simulink model "SlidingModeObserver"  (R2026b)
settings: Solver=VariableStepAuto
undefined symbols (not defined in the file or in its folder): smoCfg
libraries: AngleTracking x1
settings Model: Creator=24322  LastModifiedBy=24322

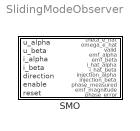
== system SlidingModeObserver ==
  SMO : Subsystem

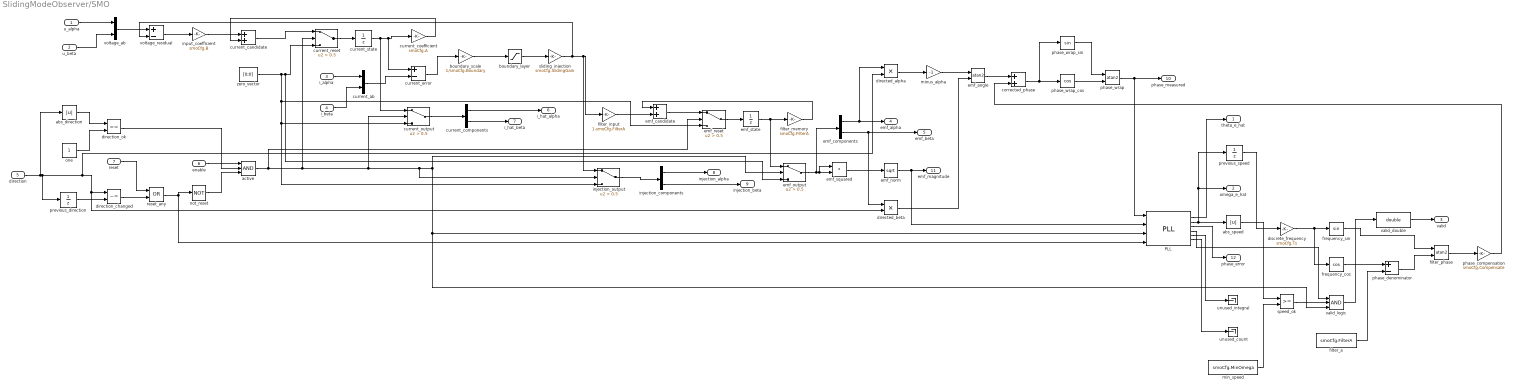
== system SlidingModeObserver/SMO ==
  u_alpha : Inport  SampleTime=smoCfg.Ts
  u_beta : Inport  Port=2  SampleTime=smoCfg.Ts
  i_alpha : Inport  Port=3  SampleTime=smoCfg.Ts
  i_beta : Inport  Port=4  SampleTime=smoCfg.Ts
  direction : Inport  Port=5  SampleTime=smoCfg.Ts
  enable : Inport  Port=6  SampleTime=smoCfg.Ts
  reset : Inport  Port=7  SampleTime=smoCfg.Ts
  PLL : AngleTracking/PLL  SystemSampleTime=-1  VariantActivationTime=update diagram  EmptyChoice=off  PassThrough=off  PassThroughVariantControl=(default)  EmptyChoiceVariantControl=(default)  AllowFlexibleInterface=on  Latency=0  AutoFrameSizeCalculation=off
  abs_direction : Abs  SaturateOnIntegerOverflow=off
  abs_speed : Abs  SaturateOnIntegerOverflow=off
  active : Logic  Inputs=3  IconShape=distinctive  AllPortsSameDT=off  OutDataTypeStr=boolean
  boundary_layer : Saturate  UpperLimit=1  LowerLimit=-1
  boundary_scale : Gain  Gain=1/smoCfg.Boundary
  corrected_phase : Sum
  current_ab : Mux  Inputs=2
  current_candidate : Sum
  current_coefficient : Gain  Gain=smoCfg.A
  current_components : Demux  Outputs=2
  current_error : Sum  Inputs=+-
  current_output : Switch  Criteria=u2 > Threshold  Threshold=0.5  SaturateOnIntegerOverflow=off  InputSameDT=off
  current_reset : Switch  Criteria=u2 > Threshold  Threshold=0.5  SaturateOnIntegerOverflow=off  InputSameDT=off
  current_state : UnitDelay  InitialCondition=[0;0]  SampleTime=smoCfg.Ts
  directed_alpha : Product  Inputs=**
  directed_beta : Product  Inputs=**
  direction_changed : RelationalOperator  Operator=~=  OutDataTypeStr=boolean  RndMeth=Simplest  InputSameDT=off
  direction_ok : RelationalOperator  Operator===  OutDataTypeStr=boolean  RndMeth=Simplest  InputSameDT=off
  discrete_frequency : Gain  Gain=smoCfg.Ts
  emf_angle : Trigonometry  Operator=atan2
  emf_candidate : Sum
  emf_components : Demux  Outputs=2
  emf_norm : Sqrt
  emf_output : Switch  Criteria=u2 > Threshold  Threshold=0.5  SaturateOnIntegerOverflow=off  InputSameDT=off
  emf_reset : Switch  Criteria=u2 > Threshold  Threshold=0.5  SaturateOnIntegerOverflow=off  InputSameDT=off
  emf_squared : DotProduct  OutDataTypeStr=Inherit: Inherit via internal rule
  emf_state : UnitDelay  InitialCondition=[0;0]  SampleTime=smoCfg.Ts
  filter_a : Constant  Value=smoCfg.FilterA
  filter_input : Gain  Gain=1-smoCfg.FilterA
  filter_memory : Gain  Gain=smoCfg.FilterA
  filter_phase : Trigonometry  Operator=atan2
  frequency_cos : Trigonometry  Operator=cos
  frequency_sin : Trigonometry
  injection_components : Demux  Outputs=2
  injection_output : Switch  Criteria=u2 > Threshold  Threshold=0.5  SaturateOnIntegerOverflow=off  InputSameDT=off
  input_coefficient : Gain  Gain=smoCfg.B
  min_speed : Constant  Value=smoCfg.MinOmega
  minus_alpha : Gain  Gain=-1
  not_reset : Logic  Operator=NOT  IconShape=distinctive  AllPortsSameDT=off  OutDataTypeStr=boolean
  one : Constant
  phase_compensation : Gain  Gain=smoCfg.Compensate
  phase_denominator : Sum  Inputs=+-
  phase_wrap : Trigonometry  Operator=atan2
  phase_wrap_cos : Trigonometry  Operator=cos
  phase_wrap_sin : Trigonometry
  previous_direction : UnitDelay  SampleTime=smoCfg.Ts
  previous_speed : UnitDelay  SampleTime=smoCfg.Ts
  reset_any : Logic  Operator=OR  IconShape=distinctive  AllPortsSameDT=off  OutDataTypeStr=boolean
  sliding_injection : Gain  Gain=smoCfg.SlidingGain
  speed_ok : RelationalOperator  OutDataTypeStr=boolean  RndMeth=Simplest  InputSameDT=off
  unused_count : Terminator
  unused_integral : Terminator
  valid_double : DataTypeConversion  OutDataTypeStr=double  SaturateOnIntegerOverflow=off  RndMeth=Floor
  valid_logic : Logic  Inputs=3  IconShape=distinctive  AllPortsSameDT=off  OutDataTypeStr=boolean
  voltage_ab : Mux  Inputs=2
  voltage_residual : Sum  Inputs=+-
  zero_vector : Constant  Value=[0;0]
  theta_e_hat : Outport
  omega_e_hat : Outport  Port=2
  valid : Outport  Port=3
  emf_alpha : Outport  Port=4
  emf_beta : Outport  Port=5
  i_hat_alpha : Outport  Port=6
  i_hat_beta : Outport  Port=7
  injection_alpha : Outport  Port=8
  injection_beta : Outport  Port=9
  phase_measured : Outport  Port=10
  emf_magnitude : Outport  Port=11
  phase_error : Outport  Port=12
  wires:
  injection_components/2 -> injection_beta/1
  current_components/2 -> i_hat_beta/1
  injection_components/1 -> injection_alpha/1
  current_components/1 -> i_hat_alpha/1
  PLL/6 -> unused_count/1
  PLL/5 -> unused_integral/1
  PLL/4 -> valid_logic/1
  PLL/3 -> phase_error/1
  PLL/2 -> omega_e_hat/1, previous_speed/1, abs_speed/1
  PLL/1 -> theta_e_hat/1
  emf_components/2 -> directed_beta/1, emf_beta/1
  emf_components/1 -> directed_alpha/1, emf_alpha/1
  valid_double/1 -> valid/1
  valid_logic/1 -> valid_double/1
  speed_ok/1 -> valid_logic/2
  min_speed/1 -> speed_ok/2
  abs_speed/1 -> speed_ok/1
  emf_norm/1 -> PLL/2, emf_magnitude/1
  phase_wrap/1 -> PLL/1, phase_measured/1
  corrected_phase/1 -> phase_wrap_sin/1, phase_wrap_cos/1
  phase_compensation/1 -> corrected_phase/2
  emf_angle/1 -> corrected_phase/1
  filter_phase/1 -> phase_compensation/1
  phase_denominator/1 -> filter_phase/2
  frequency_sin/1 -> filter_phase/1
  filter_a/1 -> phase_denominator/2
  frequency_cos/1 -> phase_denominator/1
  discrete_frequency/1 -> frequency_sin/1, frequency_cos/1
  previous_speed/1 -> discrete_frequency/1
  emf_squared/1 -> emf_norm/1
  directed_beta/1 -> emf_angle/2
  minus_alpha/1 -> emf_angle/1
  directed_alpha/1 -> minus_alpha/1
  injection_output/1 -> injection_components/1
  current_output/1 -> current_components/1
  emf_output/1 -> emf_squared/1, emf_squared/2, emf_components/1
  emf_reset/1 -> emf_state/1
  emf_candidate/1 -> emf_reset/1
  filter_input/1 -> emf_candidate/2
  filter_memory/1 -> emf_candidate/1
  emf_state/1 -> filter_memory/1, emf_output/1
  current_reset/1 -> current_state/1
  zero_vector/1 -> current_output/3, injection_output/3, emf_reset/3, current_reset/3, emf_output/3
  active/1 -> valid_logic/3, PLL/3, emf_output/2, injection_output/2, current_output/2, current_reset/2, emf_reset/2
  current_candidate/1 -> current_reset/1
  current_coefficient/1 -> current_candidate/2
  input_coefficient/1 -> current_candidate/1
  voltage_residual/1 -> input_coefficient/1
  sliding_injection/1 -> filter_input/1, injection_output/1, voltage_residual/2
  voltage_ab/1 -> voltage_residual/1
  boundary_layer/1 -> sliding_injection/1
  boundary_scale/1 -> boundary_layer/1
  current_error/1 -> boundary_scale/1
  current_ab/1 -> current_error/2
  current_state/1 -> current_error/1, current_coefficient/1, current_output/1
  not_reset/1 -> active/3
  direction_ok/1 -> active/2
  enable/1 -> active/1
  reset_any/1 -> not_reset/1, PLL/4
  direction_changed/1 -> reset_any/2
  reset/1 -> reset_any/1
  previous_direction/1 -> direction_changed/2
  one/1 -> direction_ok/2
  abs_direction/1 -> direction_ok/1
  direction/1 -> directed_beta/2, direction_changed/1, directed_alpha/2, previous_direction/1, abs_direction/1
  i_beta/1 -> current_ab/2
  i_alpha/1 -> current_ab/1
  u_beta/1 -> voltage_ab/2
  u_alpha/1 -> voltage_ab/1
  phase_wrap_cos/1 -> phase_wrap/2
  phase_wrap_sin/1 -> phase_wrap/1
